simulink model "nn"  (R2019a)
settings: Solver=ode45  StartTime=0.0  StopTime=40  RelTol=1e-3  AbsTol=1e-6
values from neighbouring files (symbols this model uses):
  u_ts = 0.001    [archneural.m]
settings Model: ExtModeTrigMode=oneshot  ExtModeArmWhenConnect=off  TunableVars=prueba  TunableVarsStorageClass=Auto  Creator=The MathWorks Inc.  LastModifiedBy=khouloud.gaaloul
settings SolverCC: AutoScaleAbsTol=off
settings DataIOCC: SaveFormat=Array  SignalLogging=off  ReturnWorkspaceOutputs=off  SignalLoggingName=sigsOut
settings OptimizationCC: BooleanDataType=off  DefaultParameterBehavior=Inlined  ExpressionDepthLimit=2147483647  InitFltsAndDblsToZero=on  LifeSpan=inf
settings DebuggingCC: SaveWithParameterizedLinksMsg=none  UnderspecifiedInitializationDetection=Classic  MergeDetectMultiDrivingBlocksExec=none  SignalResolutionControl=TryResolveAllWithWarning  MultiTaskDSMMsg=warning  MultiTaskCondExecSysMsg=none  FcnCallInpInsideContextMsg=warning  StateNameClashWarn=warning  SFUnexpectedBacktrackingDiag=warning  SFNoUnconditionalDefaultTransitionDiag=warning  SFExecutionAtInitializationDiag=none  ArithmeticOperatorsInVariantConditions=warning
settings HardwareCC: ProdBitPerPointer=32  ProdBitPerSizeT=32  ProdBitPerPtrDiffT=32  ProdLargestAtomicFloat=None  ProdIntDivRoundTo=Undefined  ProdEndianess=Unspecified  ProdWordSize=32  ProdHWDeviceType=32-bit Generic  TargetUnknown=on
settings ModelReferenceCC: PropagateSignalLabelsOutOfModel=off
settings SFSimCC: SimUseLocalCustomCode=off
settings RTWCC: TemplateMakefile=grt_vc.tmf  RTWUseLocalCustomCode=off
settings CodeAppCC: StateflowObjectComments=on
settings GRTTargetCC: TargetFcnLib=ansi_tfl_tmw.mat  TargetLangStandard=C89/C90 (ANSI)  GeneratePreprocessorConditionals=Disable all  CombineOutputUpdateFcns=off  GRTInterface=on
settings ConfigComp: CovMetricSettings=dw  CovHtmlReporting=on  CovSaveCumulativeToWorkspaceVar=on  CovSaveSingleToWorkspaceVar=on  CovExternalEMLEnable=off

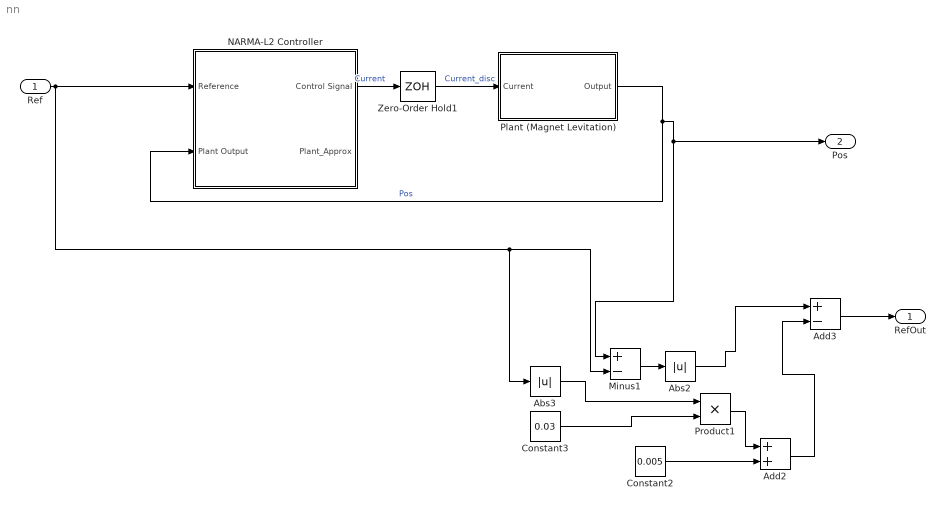
== system nn ==
  Ref : Inport  Interpolate=off
  Abs2 : Abs
  Abs3 : Abs
  Add2 : Sum
  Add3 : Sum  Inputs=+-
  Constant2 : Constant  Value=0.005
  Constant3 : Constant  Value=0.03  VectorParams1D=off
  Minus1 : Sum  Inputs=+-
  NARMA-L2 Controller : Subsystem  mask(NARMA-L2 Controller){Ts=0.01, S1=9, Ni=3, Nj=2, sim_file=ballrepel0, trainfun=trainlm, Use_validation=1, Use_Testing=1, max_i=4, min_i=-1, max_i_int=1, min_i_int=0.1, sam_training=10000, epochs=100, minp=-0.97682887932966278033, maxp=3.9954019738068033973, mint=0.0012713472471279200528, maxt=3.9954019738068033973, Normalize=1, IW1_1=[2.8569160539166240653 3.855137973617931646 2.4478436741338867044 0.86889986713150191289;0.86019748624118552716 -0.76099748761653862594 0.12978383283599650988 -0.032681949683702651854;-0.61268951567451579443 -1.3546538767805089698 -1.0357145918607806312 -2.2450213565212968625;-0.61363639390594604262 3.6302797918127760468 -2.9742392265006136753 3.7505205510025696469;8.2159425419552984948 -0.34781842703357196411 -0.63990978222347083548 3.2203753164455033442;-0.55585558555235048406 1.7347260034225613357 -0.48782067399191109125 0.15519292550861990554;0.14490936608588075862 0.091344996887225110571 -1.9999177921909609967 -1.7398058021589537514;-0.011364174849476511159 0.17210174153872684344 -0.063003341331735851494 0.016356680939399299846;1.9115353490253352842 -1.6928290742800000679 0.26139115964517828372 -0.083521590880859600259], IW3_2=[2.094012153469472004 4.1391617494602943594 0.46017743638858904509 1.4212453617040687881;-0.8698291152927356551 -0.91216393263270156844 -1.7725276755524563832 -1.8256681774546807961;-1.5212626080129232342 -1.9638393468584769419 -0.13083206166844379981 0.69514443101461376173;1.1067100747068669975 1.1077222299712199405 -1.6499992245985941608 -0.10283142888325141895;1.7627456897433946281 0.12387727106338465577 -0.74345872574560734058 1.3295242695796243293;1.3902623706994512442 1.2486843128494045096 0.60100357220348832321 1.8703374952532536568;-1.2652620294004319756 -0.81003971518970829813 0.35904126229892613376 -2.3590512744589045013;-1.7962091138833455872 0.33004248956449860897 1.1996735804361835509 -0.75846441756669458201;1.6085665816521634852 -0.65960011993077061199 2.0409314507416924656 1.300834198719902135], IW5_3=-0.86130216008060445088, LW2_1=[5.755548244449743792e-05 2.1941017287714528194 -0.00044492281828180146918 -0.00039237971120205448854 1.8234323877817898572e-06 0.042708432151687514278 0.00025330049100551882673 4.7927194580095164866 0.41991364122019325666], LW4_3=[1.1796229157074380467 1.4349048600431937306 -0.8972572979998952869 -2.3386270416842869224 -0.096692942439327439486 -0.63438599215078772531 -2.7379194644695021843 3.0145214892072624835 2.1741978843496214679], LW5_4=0.59967978592905768487, LW6_5=0.00041169382628446888304, LW6_2=0.99216750753278892816, B1=[-2.0540485030510766684;-0.2820456548276839559;-1.4224984046874724619;0.011980000365264734455;-3.2833055176157808219;1.1020848049883287256;2.2616940700361274352;-0.14165422591960777354;1.0889769241125049071], B2=0.90790507647934137747, B3=[-0.99822473976112757743;-1.1258457923320430716;1.0030562696131117839;3.6020655513043440266;-0.0251859643674823587;1.2763936285299730677;-2.2740100652873409537;-3.0720977283302817185;1.7835104510380932474], B4=0.8636776698074994929, Limit_output=1, min_output=0, max_output=Inf, Use_Previous_Weights=1}
      mask prompts: Ts "Sample time"; trainfun "Training function"
      mask help: NARMA-L2 Controller. You first train a neural network model of the plant to be controlled. The controller is a rearrangement of the trained plant model. Double-click the NARMA-L2 Controller block to begin the plant training.
      mask init:
      | xl = [0    .4   NaN  .33  .55   .55  .33  .33  NaN .80  .92 .92];
      | yl = [.95 .95 NaN  .75  .75   .55  .55  .75  NaN  .95 .95 .65];
      | x2 = [0    .43 NaN .45 .45    NaN .92 1.2 NaN .63 .85 .85 .63 .63 ];
      | y2 = [.39 .39 NaN  .41 .55   NaN .65 .65 NaN .75 .75  .55  .55  .75];
      | x3 = [.45 .45 NaN .42 .45 .48  NaN .33 .4 .33];
      | y3 = [.75 .90 NaN .83 .90 .83  NaN  .98 .95 .92];
      | x4 = [.75 .75 NaN .72 .75 .78  NaN  .5 .7 NaN .63 .7 .63];
      | y4 = [.75 .90 NaN .83 .90 .83  NaN .95 .95 NaN .98 .95 .92];
      | x5 = [.43 .43 .77 .77 .43 NaN .36 .43 .36 NaN .75 .75];
      | y5 = [.37 .41 .41 .37 .37 NaN .42 .39 .36 NaN .41 .55];
      | x6 = [.92 .92 .77 NaN .84 .77 .84];
      | y6 = [.65 .39 .39 NaN .42 .39 .36];
      | x1t=.03; y1t=.31;
      | x2t=.03; y2t=.85;
      | x8t=.03;y8t=.21;
      | x3t=.77; y3t=.53;
      | x4t=.77; y4t=.44;
      | x5t=.34; y5t=.49;
      | x6t=.58; y6t=.49;
      | 
      | 
      | t=(0:24)/24*2*pi;
      | xs = .05*cos(t);
      | ys = .05*sin(t);
      | xs1=xs+.45;
      | ys1=ys+.95;
      | xs2=xs+.75;
      | ys2=ys+.95;
      settings: OpenFcn=nncontrolutil('nnident','',gcbh,gcb,'narma_l2');
      mask TypeOptions trainfun: trainbfg | trainbr  | traincgb | traincgf | traincgp | traingd | traingdm | traingda | traingdx | trainlm  | trainoss | trainrp  | trainscg
      mask Display:
      | plot([[xl NaN x2]*.9-.075 ], [[yl  NaN y2]*.9-.1 ]);
      | plot([[x3 NaN xs1 NaN xs2]*.9-.075 ], [[y3 NaN ys1 NaN ys2]*.9-.1 ]);
      | plot([x4 NaN x5]*.9-.075,[y4 NaN y5]*.9-.1);
      | plot([x6 NaN ]*.9-.075,[y6 NaN ]*.9-.1);
      | text(x1t,y1t,'Plant');
      | text(x8t,y8t,'Output');
      | text(x2t,y2t,'Reference');
      | text(x3t,y3t,'Control');
      | text(x4t,y4t,'Signal');
      | text(x5t,y5t,'f');
      | text(x6t,y6t,'g');
  Plant (Magnet Levitation) : Subsystem
      mask init:
      | x1=[-2 -2 2 2 -2 NaN -2 -2 2 2 -2];
      | y1=[5 4 4 5 5 NaN 2 0 0 2 2];
      | x2=[-2 -2 2 2 -2 NaN -2   2  NaN -2 2 NaN 2    4    NaN 2  4];
      | y2=[4  3  3 4  4 NaN 1.5 1  NaN 1 .5 NaN 1.5 1.5 NaN .5 .5];
      | x1t = -.5 ; y1t = 4.4;
      | x2t = -.5; y2t = 3.4;
      mask Display:
      | plot([-10],[0],[10],[5]);
      | plot([x1 NaN x2],[y1 NaN y2]);
      | text(x1t,y1t,'N')
      | text(x2t,y2t,'S')
  Product1 : Product
  Zero-Order Hold1 : ZeroOrderHold  SampleTime=u_ts
  RefOut : Outport
  Pos : Outport  Port=2
  wires:
  NARMA-L2 Controller/1(Control Signal) -> Zero-Order Hold1/1  "Current"
  Zero-Order Hold1/1 -> Plant (Magnet Levitation)/1(Current)  "Current_disc"
  Minus1/1 -> Abs2/1
  Add2/1 -> Add3/2
  Plant (Magnet Levitation)/1(Output) -> NARMA-L2 Controller/2(Plant Output), Pos/1, Minus1/1  "Pos"
  Ref/1 -> NARMA-L2 Controller/1(Reference), Abs3/1, Minus1/2
  Abs3/1 -> Product1/1
  Add3/1 -> RefOut/1
  Constant3/1 -> Product1/2
  Constant2/1 -> Add2/2
  Abs2/1 -> Add3/1
  Product1/1 -> Add2/1

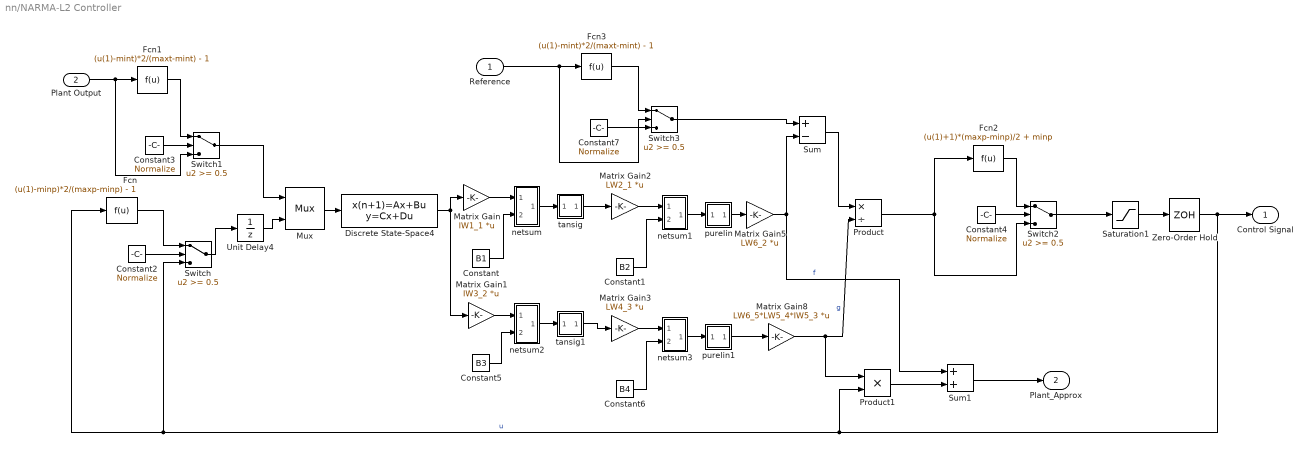
== system nn/NARMA-L2 Controller ==
  Reference : Inport
  Plant Output : Inport  Port=2
  Constant : Constant  Value=B1
  Constant1 : Constant  Value=B2
  Constant{2..4,7} (4 alike) : Constant  Value=Normalize
  Constant5 : Constant  Value=B3
  Constant6 : Constant  Value=B4
  Discrete State-Space4 : DiscreteStateSpace  A=blkdiag([zeros(1,Nj-1);eye(Nj-2,Nj-2) zeros(Nj-2,1)],[zeros(1,Ni-1);eye(Ni-2,Ni-2) zeros(Ni-2,1)])  B=blkdiag(eye(Nj-1,1),eye(Ni-1,1))  C=blkdiag([zeros(1,Nj-1);eye(Nj-1,Nj-1)],[zeros(eye(double(Ni>1)),Ni-1);eye(Ni-2,Ni-1)])  D=blkdiag([1;zeros(Nj-1,1)],[eye(double(Ni>1));zeros(Ni-2,1)])  SampleTime=Ts
  Fcn : Fcn  Expr=(u(1)-minp)*2/(maxp-minp) - 1
  Fcn1 : Fcn  Expr=(u(1)-mint)*2/(maxt-mint) - 1
  Fcn2 : Fcn  Expr=(u(1)+1)*(maxp-minp)/2 + minp
  Fcn3 : Fcn  Expr=(u(1)-mint)*2/(maxt-mint) - 1
  Matrix Gain : Gain  Gain=IW1_1  Multiplication=Matrix(K*u)  SaturateOnIntegerOverflow=on  OutDataTypeStr=Inherit: Same as input  ParamDataTypeStr=Inherit: Same as input
  Matrix Gain1 : Gain  Gain=IW3_2  Multiplication=Matrix(K*u)  SaturateOnIntegerOverflow=on  OutDataTypeStr=Inherit: Same as input  ParamDataTypeStr=Inherit: Same as input
  Matrix Gain2 : Gain  Gain=LW2_1  Multiplication=Matrix(K*u)  SaturateOnIntegerOverflow=on  OutDataTypeStr=Inherit: Same as input  ParamDataTypeStr=Inherit: Same as input
  Matrix Gain3 : Gain  Gain=LW4_3  Multiplication=Matrix(K*u)  SaturateOnIntegerOverflow=on  OutDataTypeStr=Inherit: Same as input  ParamDataTypeStr=Inherit: Same as input
  Matrix Gain5 : Gain  Gain=LW6_2  Multiplication=Matrix(K*u)  SaturateOnIntegerOverflow=on  OutDataTypeStr=Inherit: Same as input  ParamDataTypeStr=Inherit: Same as input
  Matrix Gain8 : Gain  Gain=LW6_5*LW5_4*IW5_3  Multiplication=Matrix(K*u)  SaturateOnIntegerOverflow=on  OutDataTypeStr=Inherit: Same as input  ParamDataTypeStr=Inherit: Same as input
  Mux : Mux  Inputs=2
      settings: DisplayOption=signals
  Product : Product  Inputs=*/  SaturateOnIntegerOverflow=on  InputSameDT=on  OutDataTypeStr=Inherit: Same as first input
  Product1 : Product  SaturateOnIntegerOverflow=on  InputSameDT=on  OutDataTypeStr=Inherit: Same as first input
  Saturation1 : Saturate  UpperLimit=max_i  LowerLimit=min_i  ZeroCross=off
  Sum : Sum  Inputs=+-  SaturateOnIntegerOverflow=on  InputSameDT=on  OutDataTypeStr=Inherit: Same as first input
  Sum1 : Sum  SaturateOnIntegerOverflow=on  InputSameDT=on  OutDataTypeStr=Inherit: Same as first input
  Switch{,1..3} (4 alike) : Switch  Threshold=0.5  ZeroCross=off  SaturateOnIntegerOverflow=on  InputSameDT=on
  Unit Delay4 : UnitDelay  SampleTime=Ts  HasFrameUpgradeWarning=on
  Zero-Order Hold : ZeroOrderHold  SampleTime=Ts
  netsum : Subsystem
      mask Display: disp('+')
  netsum1 : Subsystem
      mask Display: disp('+')
  netsum2 : Subsystem
      mask Display: disp('+')
  netsum3 : Subsystem
      mask Display: disp('+')
  purelin : Subsystem
      mask Display: plot([-1 1],[0 0],[-1 1],[-1 1])
  purelin1 : Subsystem
      mask Display: plot([-1 1],[0 0],[-1 1],[-1 1])
  tansig : Subsystem
      mask Display: plot([-1 1],[0 0],[-1 -.9 -.8 -.7 -.6 -.5 -.4 -.3 -.2 -.1 0 .1 .2 .3 .4 .5 .6 .7 .8 .9 1],2./(1+exp(-8*[-1 -.9 -.8 -.7 -.6 -.5 -.4 -.3 -.2 -.1 0 .1 .2 .3 .4 .5 .6 .7 .8 .9 1]))-1)
  tansig1 : Subsystem
      mask Display: plot([-1 1],[0 0],[-1 -.9 -.8 -.7 -.6 -.5 -.4 -.3 -.2 -.1 0 .1 .2 .3 .4 .5 .6 .7 .8 .9 1],2./(1+exp(-8*[-1 -.9 -.8 -.7 -.6 -.5 -.4 -.3 -.2 -.1 0 .1 .2 .3 .4 .5 .6 .7 .8 .9 1]))-1)
  Control Signal : Outport
  Plant_Approx : Outport  Port=2
  wires:
  Constant3/1 -> Switch1/2
  Fcn1/1 -> Switch1/1
  Plant Output/1 -> Fcn1/1, Switch1/3
  netsum1/1(Out1) -> purelin/1(n)
  Constant1/1 -> netsum1/2(In2)
  Matrix Gain2/1 -> netsum1/1(In1)
  netsum/1(Out1) -> tansig/1(n)
  Constant/1 -> netsum/2(In2)
  tansig/1(a) -> Matrix Gain2/1
  Matrix Gain/1 -> netsum/1(In1)
  netsum3/1(Out1) -> purelin1/1(n)
  Constant6/1 -> netsum3/2(In2)
  Matrix Gain3/1 -> netsum3/1(In1)
  netsum2/1(Out1) -> tansig1/1(n)
  Constant5/1 -> netsum2/2(In2)
  tansig1/1(a) -> Matrix Gain3/1
  Matrix Gain1/1 -> netsum2/1(In1)
  purelin/1(a) -> Matrix Gain5/1
  Matrix Gain5/1 -> Sum/2, Sum1/1  "f"
  Sum/1 -> Product/1
  purelin1/1(a) -> Matrix Gain8/1
  Matrix Gain8/1 -> Product1/1, Product/2  "g"
  Constant7/1 -> Switch3/2
  Fcn3/1 -> Switch3/1
  Reference/1 -> Fcn3/1, Switch3/3
  Switch3/1 -> Sum/1
  Switch1/1 -> Mux/1
  Mux/1 -> Discrete State-Space4/1
  Discrete State-Space4/1 -> Matrix Gain/1, Matrix Gain1/1
  Zero-Order Hold/1 -> Control Signal/1, Product1/2, Fcn/1, Switch/3  "u"
  Fcn/1 -> Switch/1
  Constant2/1 -> Switch/2
  Unit Delay4/1 -> Mux/2
  Switch/1 -> Unit Delay4/1
  Saturation1/1 -> Zero-Order Hold/1
  Product/1 -> Fcn2/1, Switch2/3
  Constant4/1 -> Switch2/2
  Switch2/1 -> Saturation1/1
  Fcn2/1 -> Switch2/1
  Product1/1 -> Sum1/2
  Sum1/1 -> Plant_Approx/1

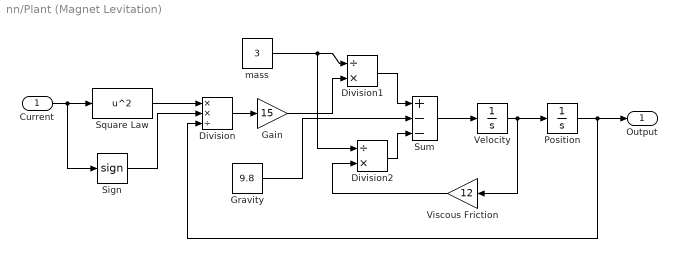
== system nn/Plant (Magnet Levitation) ==
  Current : Inport
  Division : Product  Inputs=**/  SaturateOnIntegerOverflow=on  InputSameDT=on  OutDataTypeStr=Inherit: Same as first input
  Division1 : Product  Inputs=/*  SaturateOnIntegerOverflow=on  InputSameDT=on  OutDataTypeStr=Inherit: Same as first input
  Division2 : Product  Inputs=/*  SaturateOnIntegerOverflow=on  InputSameDT=on  OutDataTypeStr=Inherit: Same as first input
  Gain : Gain  Gain=15  SaturateOnIntegerOverflow=on  OutDataTypeStr=Inherit: Same as input  ParamDataTypeStr=Inherit: Same as input
  Gravity : Constant  Value=9.8
  Position : Integrator  InitialCondition=.5  ZeroCross=off
  Sign : Signum  ZeroCross=off
  Square Law : Fcn  Expr=u^2
  Sum : Sum  Inputs=|+--  SaturateOnIntegerOverflow=on  InputSameDT=on  OutDataTypeStr=Inherit: Same as first input
  Velocity : Integrator  ZeroCross=off
  Viscous Friction : Gain  Gain=12  SaturateOnIntegerOverflow=on  OutDataTypeStr=Inherit: Same as input  ParamDataTypeStr=Inherit: Same as input
  mass : Constant  Value=3
  Output : Outport
  wires:
  Square Law/1 -> Division/1
  Division/1 -> Gain/1
  Gravity/1 -> Sum/2
  Velocity/1 -> Position/1, Viscous Friction/1
  Sum/1 -> Velocity/1
  Gain/1 -> Division1/2
  Division1/1 -> Sum/1
  mass/1 -> Division1/1, Division2/1
  Viscous Friction/1 -> Division2/2
  Division2/1 -> Sum/3
  Current/1 -> Square Law/1, Sign/1
  Position/1 -> Output/1, Division/3
  Sign/1 -> Division/2

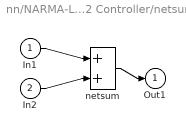
== system nn/NARMA-L2 Controller/netsum ==
  In1 : Inport
  In2 : Inport  Port=2
  netsum : Sum  Inputs=2  SaturateOnIntegerOverflow=on  InputSameDT=on  OutDataTypeStr=Inherit: Same as first input
  Out1 : Outport
  wires:
  In1/1 -> netsum/1
  In2/1 -> netsum/2
  netsum/1 -> Out1/1

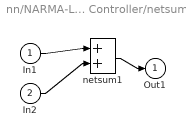
== system nn/NARMA-L2 Controller/netsum1 ==
  In1 : Inport
  In2 : Inport  Port=2
  netsum1 : Sum  Inputs=2  SaturateOnIntegerOverflow=on  InputSameDT=on  OutDataTypeStr=Inherit: Same as first input
  Out1 : Outport
  wires:
  In1/1 -> netsum1/1
  In2/1 -> netsum1/2
  netsum1/1 -> Out1/1

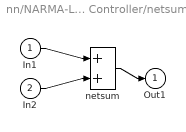
== system nn/NARMA-L2 Controller/netsum2 ==
  In1 : Inport
  In2 : Inport  Port=2
  netsum : Sum  Inputs=2  SaturateOnIntegerOverflow=on  InputSameDT=on  OutDataTypeStr=Inherit: Same as first input
  Out1 : Outport
  wires:
  In1/1 -> netsum/1
  In2/1 -> netsum/2
  netsum/1 -> Out1/1

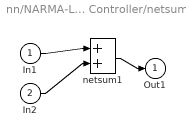
== system nn/NARMA-L2 Controller/netsum3 ==
  In1 : Inport
  In2 : Inport  Port=2
  netsum1 : Sum  Inputs=2  SaturateOnIntegerOverflow=on  InputSameDT=on  OutDataTypeStr=Inherit: Same as first input
  Out1 : Outport
  wires:
  In1/1 -> netsum1/1
  In2/1 -> netsum1/2
  netsum1/1 -> Out1/1

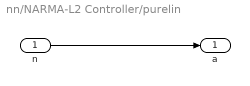
== system nn/NARMA-L2 Controller/purelin ==
  n : Inport
  a : Outport
  wires:
  n/1 -> a/1

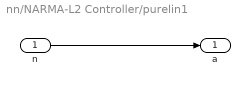
== system nn/NARMA-L2 Controller/purelin1 ==
  n : Inport
  a : Outport
  wires:
  n/1 -> a/1

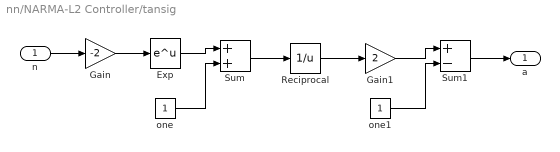
== system nn/NARMA-L2 Controller/tansig ==
  n : Inport
  Exp : Math  SaturateOnIntegerOverflow=on
  Gain : Gain  Gain=-2  SaturateOnIntegerOverflow=on  OutDataTypeStr=Inherit: Same as input  ParamDataTypeStr=Inherit: Same as input
  Gain1 : Gain  Gain=2  SaturateOnIntegerOverflow=on  OutDataTypeStr=Inherit: Same as input  ParamDataTypeStr=Inherit: Same as input
  Reciprocal : Math  Operator=reciprocal  SaturateOnIntegerOverflow=on
  Sum : Sum  SaturateOnIntegerOverflow=on  InputSameDT=on  OutDataTypeStr=Inherit: Same as first input
  Sum1 : Sum  Inputs=+-  SaturateOnIntegerOverflow=on  InputSameDT=on  OutDataTypeStr=Inherit: Same as first input
  one : Constant
  one1 : Constant
  a : Outport
  wires:
  n/1 -> Gain/1
  Gain/1 -> Exp/1
  Exp/1 -> Sum/1
  one/1 -> Sum/2
  Sum/1 -> Reciprocal/1
  Reciprocal/1 -> Gain1/1
  Gain1/1 -> Sum1/1
  one1/1 -> Sum1/2
  Sum1/1 -> a/1

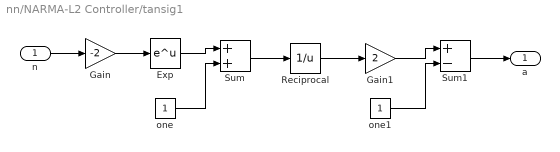
== system nn/NARMA-L2 Controller/tansig1 ==
  n : Inport
  Exp : Math  SaturateOnIntegerOverflow=on
  Gain : Gain  Gain=-2  SaturateOnIntegerOverflow=on  OutDataTypeStr=Inherit: Same as input  ParamDataTypeStr=Inherit: Same as input
  Gain1 : Gain  Gain=2  SaturateOnIntegerOverflow=on  OutDataTypeStr=Inherit: Same as input  ParamDataTypeStr=Inherit: Same as input
  Reciprocal : Math  Operator=reciprocal  SaturateOnIntegerOverflow=on
  Sum : Sum  SaturateOnIntegerOverflow=on  InputSameDT=on  OutDataTypeStr=Inherit: Same as first input
  Sum1 : Sum  Inputs=+-  SaturateOnIntegerOverflow=on  InputSameDT=on  OutDataTypeStr=Inherit: Same as first input
  one : Constant
  one1 : Constant
  a : Outport
  wires:
  n/1 -> Gain/1
  Gain/1 -> Exp/1
  Exp/1 -> Sum/1
  one/1 -> Sum/2
  Sum/1 -> Reciprocal/1
  Reciprocal/1 -> Gain1/1
  Gain1/1 -> Sum1/1
  one1/1 -> Sum1/2
  Sum1/1 -> a/1
